simulink model "AutoSarNm"  (R2022b)
settings: Solver=FixedStepDiscrete  StartTime=0.0  StopTime=inf  FixedStep=0.01  RelTol=1e-3
PreLoadFcn:
  | canMessageBusType;
  | canFDMessageBusType;
values from neighbouring files (symbols this model uses):
  AUROSAR_NM_CANWAKEUP_ENABLE = 1.0    [AutoSarNm.sldd]
  AUROSAR_NM_MODEL_RUN_STEP = 10.0    [AutoSarNm.sldd]
  AUROSAR_NM_RDY2SLP_ENABLE = 0.0    [AutoSarNm.sldd]
  AUROSAR_NM_UDS_OVERTIME = 5000.0    [AutoSarNm.sldd]
  CAN_ID_VEH_RX_NM = 418316033    [AutoSarNm.sldd]
  CAN_ID_VEH_TX_NM = 536870910.0    [AutoSarNm.sldd]
  CANNM_BSM_WAITSLP_TIME = 500.0    [AutoSarNm.sldd]
  CANNM_IMMEDIATE_CYCLE_TIME = 20.0    [AutoSarNm.sldd]
  CANNM_IMMEDIATE_TRANSMISSION_COUNT = 10.0    [AutoSarNm.sldd]
  CANNM_MSG_CYCLE_TIME = 1000.0    [AutoSarNm.sldd]
  CANNM_NM_TIMEOUT_TIME = 2500.0    [AutoSarNm.sldd]
  CANNM_REPEAT_MEG_TIME = 3300.0    [AutoSarNm.sldd]
  CANNM_WAIT_BUS_SLEEP_TIME = 1500.0    [AutoSarNm.sldd]
libraries: simulink x7, canfdmsglib x2
PreSaveFcn:
  | filename = 'AutoSarNm';
  | dictionaryObj  = Simulink.data.dictionary.open([filename,'.sldd']);
  | saveChanges(dictionaryObj);
  | close(dictionaryObj);
  | disp([filename,'.sldd 已保存']);
settings Model: DataDictionary=AutoSarNm.sldd  Creator=Ligoo  LastModifiedBy=CASTORICE
settings DataIOCC: SaveOutput=off  SignalLogging=off  DSMLogging=off  SaveTime=off  ReturnWorkspaceOutputs=off
settings OptimizationCC: DefaultParameterBehavior=Inlined  DefaultUnderspecifiedDataType=single  EnableMemcpy=off  ActiveStateOutputEnumStorageType=uint16  ZeroExternalMemoryAtStartup=off  ZeroInternalMemoryAtStartup=off  NoFixptDivByZeroProtection=on  EfficientFloat2IntCast=on  LifeSpan=Inf  MaxStackSize=200  OptimizeBlockOrder=speed  DifferentSizesBufferReuse=on  EfficientTunableParamExpr=on
settings DebuggingCC: SignalInfNanChecking=error  SignalRangeChecking=warning  AlgebraicLoopMsg=error  MergeDetectMultiDrivingBlocksExec=none  TasksWithSamePriorityMsg=error  IntegerOverflowMsg=error  UnconnectedInputMsg=error  UnconnectedOutputMsg=error  UnconnectedLineMsg=error  UniqueDataStoreMsg=warning  ModelReferenceIOMsg=error  ModelReferenceVersionMismatchMessage=error  StateNameClashWarn=warning  SFUnexpectedBacktrackingDiag=warning  SFNoUnconditionalDefaultTransitionDiag=warning  SFUndirectedBroadcastEventsDiag=error  IntegerSaturationMsg=error
settings HardwareCC: ProdBitPerPointer=32  ProdBitPerSizeT=32  ProdBitPerPtrDiffT=32  ProdLargestAtomicInteger=Long  ProdWordSize=32  ProdLongLongMode=on  ProdHWDeviceType=ARM Compatible->ARM 7
settings ModelReferenceCC: EnableRefExpFcnMdlSchedulingChecks=on
settings SFSimCC: SimCustomHeaderCode="#include \"NMmain.h\""  SimUserSources=NMmain.c  MATLABDynamicMemAlloc=off
settings RTWCC: Description=Embedded Coder  SystemTargetFile=ert.tlc  GenCodeOnly=on  TemplateMakefile=ert_default_tmf  GenerateReport=on  RTWUseSimCustomCode=on  CustomHeaderCode="#include \"NMmain.h\""  CustomSource=NMmain.c  Toolchain=LCC-win64 v2.4.1 | gmake (64-bit Windows)  IncludeHyperlinkInReport=on  LaunchReport=on  GenerateTraceInfo=on  GenerateTraceReport=on  GenerateTraceReportSl=on  GenerateTraceReportSf=on  GenerateTraceReportEml=on
settings CodeAppCC: ForceParamTrailComments=on  IgnoreCustomStorageClasses=off  OperatorAnnotations=on  SimulinkDataObjDesc=on  SFDataObjDesc=on  MATLABFcnDesc=on  CustomSymbolStrUtil=$R$N$C  InsertBlockDesc=on  MATLABSourceComments=on
settings ERTTargetCC: MultiwordLength=2048  ConcurrentExecutionCompliant=off  IncludeMdlTerminateFcn=off  SuppressErrorStatus=on  SupportAbsoluteTime=off  SupportNonFinite=off  SupportComplex=off  ModelStepFunctionPrototypeControlCompliant=off  CPPClassGenCompliant=off  ArrayLayout=Row-major  GenerateASAP2=on  InlinedParameterPlacement=NonHierarchical  ERTCustomFileTemplate=example_file_process.tlc
settings ConfigComp: CovSaveCumulativeToWorkspaceVar=on  CovSaveSingleToWorkspaceVar=on  CovExternalEMLEnable=off  DVTestSuiteOptimization=CombinedObjectives (Nonlinear Extended)  DVDetectActiveLogic=on  DVModelReferenceHarness=on  DVHarnessSource=Signal Editor

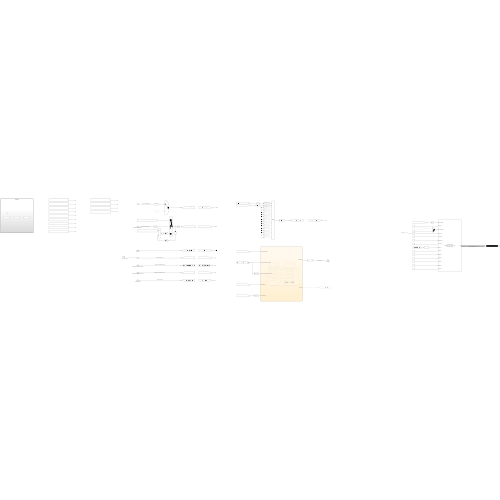
[thumbnail: Simulink's stored preview of the top-level diagram]
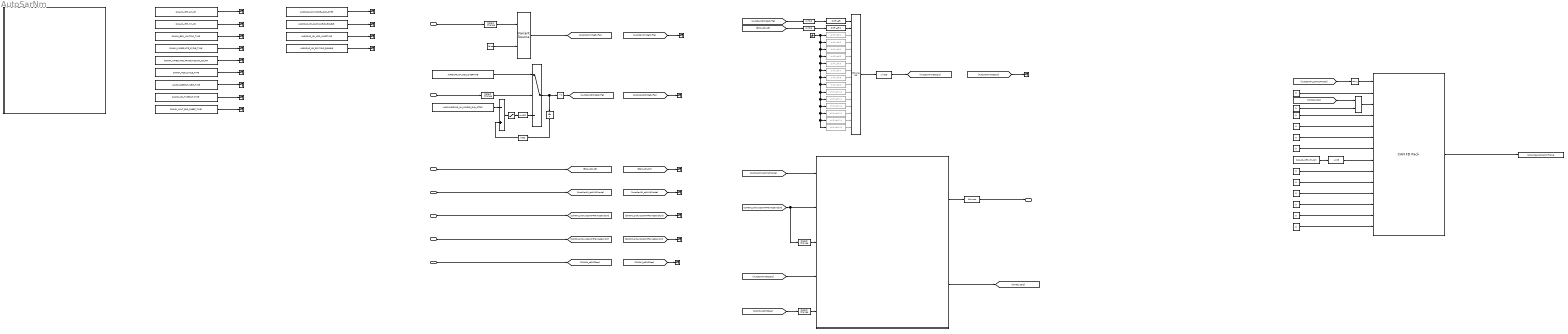
== system AutoSarNm ==
  note: 0:被动唤醒
      | 1:主动唤醒
      | 0xFF:未探测到唤醒源
  note: 分段网络管理，不支持
  AutoSarNM_cntNmMsgRxCnt : Inport
  AutoSarNM_cntUDSMsgRxCnt : Inport  Port=2
  BSW_stKL15 : Inport  Port=3
  AutoSarNM_stWKUPMode : Inport  Port=4
  CANNM_cntAuroSarNMFrameSendCnt : Inport  Port=5
  CANNM_cntAuroSarNMFrameRecvCnt : Inport  Port=6
  CANNM_stRMSReq : Inport  Port=7
  Add : Sum  Inputs=-+  OutDataTypeStr=int32
  Bitwise OR : simulink/Logic and Bit Operations/Bitwise Operator  logicop=OR  UseBitMask=off  NumInputPorts=16  BitMask=bin2dec('11011001')  BitMaskRealWorld=Stored Integer
      settings: LibrarySourceBlock=|
      | simulink/Quick Insert/Logic and Bit
      | Operations/Bitwise OR
  CAN FD Pack : canfdmsglib/CAN FD Pack  MsgList=(none)  MsgName=AutoSarNM  ProtocolMode=CAN FD  MsgIDType=Extended (29-bit identifier)  MsgIdentifier=CAN_ID_VEH_TX_NM  MsgLength=8  Remote=off  BRSSwitch=on  ApplyMinMax=off  SignalInfo={ 'CBV_ActWKUP', '12', '1', 'BE', 'unsigned', 'Standard', '0', '1', '0', '-Inf', 'Inf'; 'CBV_CID', '9', '2', 'BE', 'unsigned', 'Standard', '0', '1', '0', '-Inf', 'Inf'; 'CBV_NmSlpRdy', '11', '1', 'BE', 'unsigned', 'Standard', '0', '1', '0', '-Inf', 'Inf'; 'CBV_PNI', '14', '1', 'BE', 'unsigned', 'Standard', '0', '1', '0', '-Inf', 'Inf'; 'CBV_RESV_1', '13', '1', 'BE', 'unsigned', 'Standard', '0', '1', '0', '-Inf', 'Inf'; 'CBV_RESV_2', '15', '1', 'BE', 'unsigned', 'Standard', '0', '1', '0', '-Inf', 'Inf'; 'CBV_RMR', '8', '1', 'BE', 'unsigned', 'Standard', '0', '1', '0', '-Inf', 'Inf'; 'SourceID', '0', '8', 'BE', 'unsigned', 'Standard', '0', '1', '0', '-Inf', 'Inf'; 'UseData1', '16', '8', 'BE', 'unsigned', 'Standard', '0', '1', '0', '-Inf', 'Inf'; 'UseData2', '24', '8', 'BE', 'unsigned', 'Standard', '0', '1', '0', '-Inf', 'Inf'; 'UseData3', '32', '8', 'BE', 'unsigned', 'Standard', '0', '1', '0', '-Inf', 'Inf'; 'UseData4', '40', '8', 'BE', 'unsigned', 'Standard', '0', '1', '0', '-Inf', 'Inf'; 'UseData5', '48', '8', 'BE', 'unsigned', 'Standard', '0', '1', '0', '-Inf', 'Inf'; 'UseData6', '56', '8', 'BE', 'unsigned', 'Standard', '0', '1', '0', '-Inf', 'Inf' }
      settings: DataFormat=manually specified signals
  Chart : Stateflow chart  TreatAsAtomicUnit=on
  Compare To Constant : simulink/Logic and Bit Operations/Compare To Constant  relop=~=  const=uint32(0)  OutDataTypeStr=boolean
  Compare To Constant1 : simulink/Logic and Bit Operations/Compare To Constant  relop===  const=1  OutDataTypeStr=uint8
  Constant : Constant  Value=AUROSAR_NM_CANWAKEUP_ENABLE
  Constant1 : Constant  Value=AUROSAR_NM_MODEL_RUN_STEP
  Constant{9..12,14..20,29} (12 alike) : Constant  Value=0  OutDataTypeStr=uint8
  Constant13 : Constant  Value=AUROSAR_NM_RDY2SLP_ENABLE
  Constant2 : Constant  Value=false  OutDataTypeStr=boolean
  Constant21 : Constant  Value=CAN_ID_VEH_TX_NM
  Constant22 : Constant  Value=CANNM_BSM_WAITSLP_TIME
  Constant23 : Constant  Value=CANNM_IMMEDIATE_CYCLE_TIME
  Constant24 : Constant  Value=CANNM_IMMEDIATE_TRANSMISSION_COUNT
  Constant25 : Constant  Value=CANNM_MSG_CYCLE_TIME
  Constant26 : Constant  Value=CANNM_REPEAT_MEG_TIME
  Constant27 : Constant  Value=CANNM_NM_TIMEOUT_TIME
  Constant28 : Constant  Value=CANNM_WAIT_BUS_SLEEP_TIME
  Constant3 : Constant  Value=AUROSAR_NM_UDS_OVERTIME
  Constant4 : Constant  Value=AUROSAR_NM_UDS_OVERTIME
  Constant5 : Constant  Value=int32(AUROSAR_NM_MODEL_RUN_STEP)
  Constant7 : Constant  Value=CAN_ID_VEH_RX_NM
  Constant8 : Constant  Value=CAN_ID_VEH_TX_NM  OutDataTypeStr=uint32
  Data Store Write : DataStoreWrite  DataStoreName=CAN_msgAutoSarNmFrame  IndexOptions=Index vector (dialog)  Indices=1  OutputSizes=1
  Data Type Conversion : DataTypeConversion  OutDataTypeStr=uint16  SaturateOnIntegerOverflow=off  RndMeth=Floor
  Data Type Conversion1 : DataTypeConversion  OutDataTypeStr=Enum: AutoSarNm_Sts_Enum  SaturateOnIntegerOverflow=off  RndMeth=Floor
  Data Type Conversion2 : DataTypeConversion  OutDataTypeStr=uint16  SaturateOnIntegerOverflow=off  RndMeth=Floor
  Data Type Conversion3 : DataTypeConversion  OutDataTypeStr=uint16  SaturateOnIntegerOverflow=off  RndMeth=Floor
  Data Type Conversion4 : DataTypeConversion  OutDataTypeStr=int32  SaturateOnIntegerOverflow=off  RndMeth=Floor
  Data Type Conversion5 : DataTypeConversion  OutDataTypeStr=uint32  SaturateOnIntegerOverflow=off  RndMeth=Floor
  Data Type Conversion6 : DataTypeConversion  OutDataTypeStr=uint8  SaturateOnIntegerOverflow=off  RndMeth=Floor
  Detect Change : simulink/Logic and Bit Operations/Detect Change  vinit=0  OutDataTypeStr=boolean
  Detect Change1 : simulink/Logic and Bit Operations/Detect Change  vinit=0  OutDataTypeStr=boolean
  Detect Change2 : simulink/Logic and Bit Operations/Detect Change  vinit=0  OutDataTypeStr=uint8
  Detect Change3 : simulink/Logic and Bit Operations/Detect Change  vinit=0  OutDataTypeStr=uint8
  Ground : Ground
  Initialize Function : Subsystem  TreatAsAtomicUnit=on
  Saturation : Saturate  UpperLimit=int32(AUROSAR_NM_UDS_OVERTIME)  LowerLimit=0
  Shift Arithmetic : ArithShift  BitShiftDirection=Left
  Shift Arithmetic1 : ArithShift  BitShiftNumber=1  BitShiftDirection=Left
  Shift Arithmetic10 : ArithShift  Commented=on  BitShiftNumber=10  BitShiftDirection=Left
  Shift Arithmetic11 : ArithShift  Commented=on  BitShiftNumber=11  BitShiftDirection=Left
  Shift Arithmetic12 : ArithShift  Commented=on  BitShiftNumber=12  BitShiftDirection=Left
  Shift Arithmetic13 : ArithShift  Commented=on  BitShiftNumber=13  BitShiftDirection=Left
  Shift Arithmetic14 : ArithShift  Commented=on  BitShiftNumber=14  BitShiftDirection=Left
  Shift Arithmetic15 : ArithShift  Commented=on  BitShiftNumber=15  BitShiftDirection=Left
  Shift Arithmetic2 : ArithShift  Commented=on  BitShiftNumber=2  BitShiftDirection=Left
  Shift Arithmetic3 : ArithShift  Commented=on  BitShiftNumber=3  BitShiftDirection=Left
  Shift Arithmetic4 : ArithShift  Commented=on  BitShiftNumber=4  BitShiftDirection=Left
  Shift Arithmetic5 : ArithShift  Commented=on  BitShiftNumber=5  BitShiftDirection=Left
  Shift Arithmetic6 : ArithShift  Commented=on  BitShiftNumber=6  BitShiftDirection=Left
  Shift Arithmetic7 : ArithShift  Commented=on  BitShiftNumber=7  BitShiftDirection=Left
  Shift Arithmetic8 : ArithShift  Commented=on  BitShiftNumber=8  BitShiftDirection=Left
  Shift Arithmetic9 : ArithShift  Commented=on  BitShiftNumber=9  BitShiftDirection=Left
  Switch : Switch  Criteria=u2 > Threshold  SaturateOnIntegerOverflow=off  InputSameDT=off
  Terminator{,1..20} (21 alike) : Terminator
  Unit Delay : UnitDelay  SampleTime=-1  HasFrameUpgradeWarning=on
  Variant Source : VariantSource  VariantActivationTime=code compile
  Variant Source1 : VariantSource  VariantActivationTime=code compile
  AutoSarNM_sts : Outport
  wires:
  Constant/1 -> Terminator/1
  AutoSarNM_cntNmMsgRxCnt/1 -> Detect Change/1  "AutoSarNM_cntNmMsgRxCnt"
  Constant1/1 -> Terminator1/1
  Detect Change/1 -> Variant Source/1
  Constant2/1 -> Variant Source/2
  Variant Source/1 -> [AutoSarNmMsgRxFlg]
  [AutoSarNmMsgRxFlg] -> Terminator2/1
  AutoSarNM_cntUDSMsgRxCnt/1 -> Detect Change1/1  "AutoSarNM_cntUDSMsgRxCnt"
  Constant3/1 -> Terminator3/1
  Detect Change1/1 -> Switch/2
  Constant4/1 -> Switch/1
  Add/1 -> Saturation/1
  Switch/1 -> Compare To Constant/1, Unit Delay/1
  Unit Delay/1 -> Data Type Conversion4/1
  Constant5/1 -> Add/1
  Saturation/1 -> Data Type Conversion5/1
  Compare To Constant/1 -> [AutoSarUDSMsgRxFlg]
  [AutoSarUDSMsgRxFlg] -> Terminator4/1
  [AutoSarUDSMsgRxFlg] -> Data Type Conversion2/1
  BSW_stKL15/1 -> [BSW_stKL15]  "BSW_stKL15"
  [BSW_stKL15] -> Terminator5/1
  Shift Arithmetic/1 -> Bitwise OR/1
  Bitwise OR/1 -> Data Type Conversion/1
  [BSW_stKL15] -> Data Type Conversion3/1
  Shift Arithmetic1/1 -> Bitwise OR/2
  Ground/1 -> Shift Arithmetic15/1, Shift Arithmetic14/1, Shift Arithmetic13/1, Shift Arithmetic12/1, Shift Arithmetic11/1, Shift Arithmetic10/1, Shift Arithmetic9/1, Shift Arithmetic8/1, Shift Arithmetic7/1, Shift Arithmetic6/1, Shift Arithmetic5/1, Shift Arithmetic4/1, Shift Arithmetic3/1, Shift Arithmetic2/1
  Shift Arithmetic2/1 -> Bitwise OR/3
  Shift Arithmetic3/1 -> Bitwise OR/4
  Shift Arithmetic4/1 -> Bitwise OR/5
  Shift Arithmetic5/1 -> Bitwise OR/6
  Shift Arithmetic6/1 -> Bitwise OR/7
  Shift Arithmetic7/1 -> Bitwise OR/8
  Shift Arithmetic8/1 -> Bitwise OR/9
  Shift Arithmetic9/1 -> Bitwise OR/10
  Shift Arithmetic10/1 -> Bitwise OR/11
  Shift Arithmetic11/1 -> Bitwise OR/12
  Shift Arithmetic12/1 -> Bitwise OR/13
  Shift Arithmetic13/1 -> Bitwise OR/14
  Shift Arithmetic14/1 -> Bitwise OR/15
  Shift Arithmetic15/1 -> Bitwise OR/16
  Data Type Conversion/1 -> [AutoSarNmKeepSrc]
  [AutoSarNmKeepSrc] -> Terminator6/1
  Constant7/1 -> Terminator7/1
  Constant8/1 -> Data Type Conversion6/1
  Constant9/1 -> CAN FD Pack/4
  Constant10/1 -> CAN FD Pack/5
  Constant11/1 -> CAN FD Pack/6
  Constant12/1 -> CAN FD Pack/7
  AutoSarNM_stWKUPMode/1 -> [AutoSarNM_stWKUPMode]  "AutoSarNM_stWKUPMode"
  Constant14/1 -> CAN FD Pack/2
  Constant15/1 -> CAN FD Pack/9
  Constant16/1 -> CAN FD Pack/10
  Constant17/1 -> CAN FD Pack/11
  Constant18/1 -> CAN FD Pack/12
  Constant19/1 -> CAN FD Pack/13
  Constant20/1 -> CAN FD Pack/14
  Constant21/1 -> Terminator8/1
  Constant22/1 -> Terminator9/1
  [AutoSarNM_stWKUPMode] -> Terminator10/1
  [AutoSarNM_stWKUPMode] -> Compare To Constant1/1
  Compare To Constant1/1 -> CAN FD Pack/1
  [AutoSarNM_stWKUPMode] -> Chart/1(AutoSarNM_stWKUPMode)
  Constant23/1 -> Terminator11/1
  CANNM_cntAuroSarNMFrameSendCnt/1 -> [CANNM_cntAuroSarNMFrameSendCnt]  "CANNM_cntAuroSarNMFrameSendCnt"
  [CANNM_cntAuroSarNMFrameSendCnt] -> Terminator12/1
  [CANNM_cntAuroSarNMFrameSendCnt] -> Detect Change3/1, Chart/2(CANNM_cntAuroSarNMFrameSendCnt)
  Constant24/1 -> Terminator13/1
  CANNM_cntAuroSarNMFrameRecvCnt/1 -> [CANNM_cntAuroSarNMFrameRecvCnt]  "CANNM_cntAuroSarNMFrameRecvCnt"
  [CANNM_cntAuroSarNMFrameRecvCnt] -> Terminator14/1
  Constant25/1 -> Terminator15/1
  [AutoSarNmKeepSrc] -> Chart/4(AutoSarNmKeepSrc)
  Constant26/1 -> Terminator16/1
  Chart/1(AutoSarNM_sts) -> Data Type Conversion1/1
  CANNM_stRMSReq/1 -> [CANNM_stRMSReq]  "CANNM_stRMSReq"
  [CANNM_stRMSReq] -> Terminator17/1
  [CANNM_stRMSReq] -> Detect Change2/1
  Detect Change2/1 -> Chart/5(CANNM_stRMSReq)
  Constant27/1 -> Terminator18/1
  Constant28/1 -> Terminator19/1
  Chart/2(NmRdy2Slp) -> [NmRdy2Slp]
  Data Type Conversion1/1 -> AutoSarNM_sts/1  "AutoSarNM_sts"
  Data Type Conversion2/1 -> Shift Arithmetic/1
  Data Type Conversion3/1 -> Shift Arithmetic1/1
  Data Type Conversion4/1 -> Add/2
  Data Type Conversion5/1 -> Switch/3
  CAN FD Pack/1 -> Data Store Write/1  "CAN_msgAutoSarNmFrame"
  Data Type Conversion6/1 -> CAN FD Pack/8
  Detect Change3/1 -> Chart/3(CANNM_cntAuroSarNMFrameSendCnt_Step)
  Constant13/1 -> Terminator20/1
  Variant Source1/1 -> CAN FD Pack/3
  [NmRdy2Slp] -> Variant Source1/1
  Constant29/1 -> Variant Source1/2

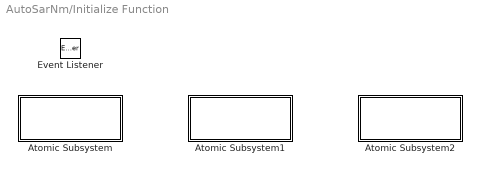
== system AutoSarNm/Initialize Function ==
  Atomic Subsystem : Subsystem  Priority=1  TreatAsAtomicUnit=on
  Atomic Subsystem1 : Subsystem  Priority=2  TreatAsAtomicUnit=on
  Atomic Subsystem2 : Subsystem  Priority=3  TreatAsAtomicUnit=on
  Event Listener : EventListener  DisableCoverage=on  EventName=reset

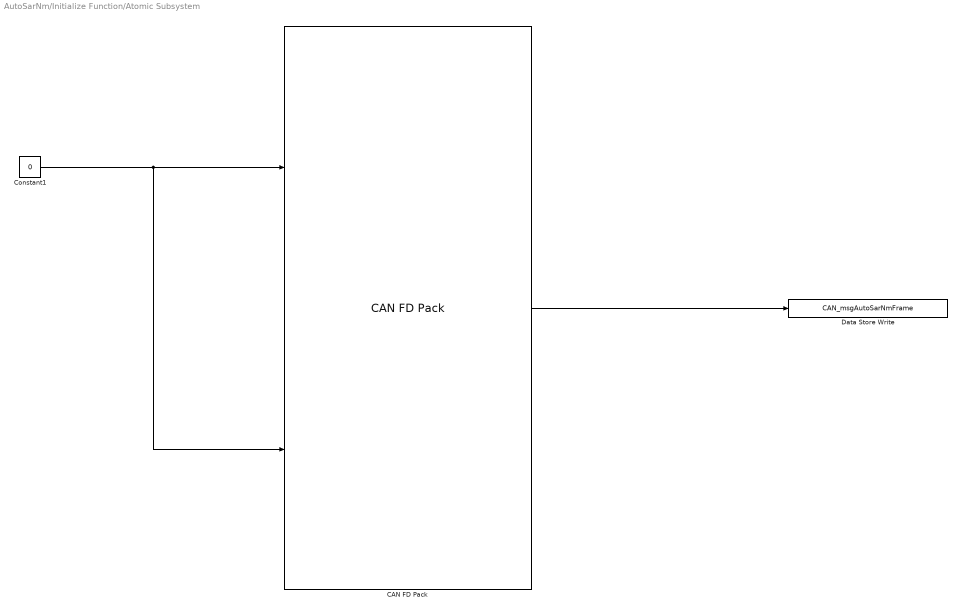
== system AutoSarNm/Initialize Function/Atomic Subsystem ==
  CAN FD Pack : canfdmsglib/CAN FD Pack  MsgList=(none)  MsgName=AutoSarNM  ProtocolMode=CAN FD  MsgIDType=Extended (29-bit identifier)  MsgIdentifier=CAN_ID_VEH_TX_NM  MsgLength=8  Remote=off  BRSSwitch=on  ApplyMinMax=off  SignalInfo={ 'Signal1', '0', '32', 'LE', 'signed', 'Standard', '0', '1', '0', '-Inf', 'Inf'; 'Signal2', '32', '32', 'LE', 'signed', 'Standard', '0', '1', '0', '-Inf', 'Inf' }
      settings: DataFormat=manually specified signals
  Constant1 : Constant  Value=0  OutDataTypeStr=uint8
  Data Store Write : DataStoreWrite  DataStoreName=CAN_msgAutoSarNmFrame  IndexOptions=Index vector (dialog)  Indices=1  OutputSizes=1
  wires:
  CAN FD Pack/1 -> Data Store Write/1
  Constant1/1 -> CAN FD Pack/2, CAN FD Pack/1

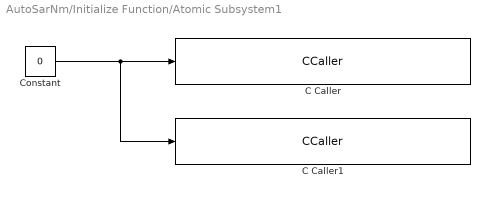
== system AutoSarNm/Initialize Function/Atomic Subsystem1 ==
  C Caller : CCaller  FunctionName=NM_SetAppMsgEnable  PortSpecificationStruct="%)30     .    * (   8    (     @         %    \"     $    !     0         %  0 \"0    $    _    07)G3F%M90  4&]R=$YA;64 4V-O<&4     26YD97@     5'EP90      4VEZ90      27-';&]B86P   X    X    !@    @    $          4    (     0    8    !         !     &    16YA8FQE   .    .     8    (    !          %    \"     $    &     0         0    !@   $5N86)L90  #@   #@    &    \"     0         !0    @    !    !0    $         $     4   !);G!U=     X    X    !@    @    &          4    (     0    $    !          D    (               .    .     8    (    !          %    \"     $    %     0         0    !0   '5I;G0X    #@   #     &    \"     0         !0    @    !     0    $         $  ! #$    .    ,     8    (    \"0(        %    \"     $    !     0         \"  $"
  C Caller1 : CCaller  FunctionName=NM_SetNmMsgEnable  PortSpecificationStruct="%)30     .    * (   8    (     @         %    \"     $    !     0         %  0 \"0    $    _    07)G3F%M90  4&]R=$YA;64 4V-O<&4     26YD97@     5'EP90      4VEZ90      27-';&]B86P   X    X    !@    @    $          4    (     0    8    !         !     &    16YA8FQE   .    .     8    (    !          %    \"     $    &     0         0    !@   $5N86)L90  #@   #@    &    \"     0         !0    @    !    !0    $         $     4   !);G!U=     X    X    !@    @    &          4    (     0    $    !          D    (               .    .     8    (    !          %    \"     $    %     0         0    !0   '5I;G0X    #@   #     &    \"     0         !0    @    !     0    $         $  ! #$    .    ,     8    (    \"0(        %    \"     $    !     0         \"  $"
  Constant : Constant  Value=0  OutDataTypeStr=uint8
  wires:
  Constant/1 -> C Caller1/1, C Caller/1

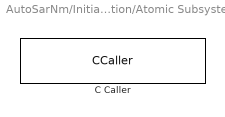
== system AutoSarNm/Initialize Function/Atomic Subsystem2 ==
  C Caller : CCaller  FunctionName=NM_BsmGetWkupMode

== stateflow chart AutoSarNm/Chart ==
  state BSM
    en:
    NM_SetNmMsgEnable(uint8(0));
    NM_SetAppMsgEnable(uint8(0));
    NM_ResetCanNmSendCnt();
    App_SendFlg = 0;
    AutoSarNM_sts = uint8(0);
    NmRdy2Slp = 0;
    NM_PbsmGetWkupMode(uint8(1));
    du:
    NM_PbsmGetWkupMode(uint8(0));
    state wait
    state wait1
      en:
      NM_EnterSleepMode();
    (default) -> BSM.wait
    BSM.wait -> wait1 : [after(CANNM_BSM_WAITSLP_TIME,msec)]
  state PBSM
    en:
    AutoSarNM_sts = uint8(1);
    NM_SetAppMsgEnable(uint8(0));
    NM_ResetCanNmSendCnt();
    NM_ResetWKUPMode();
    App_SendFlg = 0;
    NM_PbsmGetWkupMode(uint8(1));
    du:
    NM_PbsmGetWkupMode(uint8(0));
  state ALL
    state RMS
      en:
      AutoSarNM_sts = uint8(2);
      %1、上电后首帧必须是网管管理帧
      %2、被动唤醒不进入快发模式
      state Set_AppSendMode [parallel]
        settings: executionOrder=1
        state Fast
        state Slow
          en:
          NM_SetAppMsgEnable(uint8(1));
          App_SendFlg = 1;
        (default) -> ALL.RMS.Set_AppSendMode.Fast [order 1] : [App_SendFlg == 0]
        (default) -> ALL.RMS.Set_AppSendMode.Slow [order 2]
        ALL.RMS.Set_AppSendMode.Fast -> ALL.RMS.Set_AppSendMode.Slow : [CANNM_cntAuroSarNMFrameSendCnt > 0]
      state Set_NmSendMode [parallel]
        settings: executionOrder=2
        state Slow
          en:
          NM_SetNmMsgEnable(uint8(1));
          NM_SetNmMsgCycle(CANNM_MSG_CYCLE_TIME);
        state Fast
          en:
          NM_SetNmMsgCycle(CANNM_IMMEDIATE_CYCLE_TIME);
          NM_SetNmMsgEnable(uint8(1));
          NM_ResetCanNmSendCnt();
          RMSSendFrameCntDelay = CANNM_cntAuroSarNMFrameSendCnt;
        (default) -> ALL.RMS.Set_NmSendMode.Slow [order 2]
        (default) -> ALL.RMS.Set_NmSendMode.Fast [order 1] : [AutoSarNM_stWKUPMode == 0 || CANNM_stRMSReq ~= 0]
        ALL.RMS.Set_NmSendMode.Fast -> ALL.RMS.Set_NmSendMode.Slow : [CANNM_cntAuroSarNMFrameSendCnt - RMSSendFrameCntDelay >= CANNM_IMMEDIATE_TRANSMISSION_COUNT]
    state NOS
      en:
      AutoSarNM_sts = uint8(3);
    state RSS
      en:
      AutoSarNM_sts = uint8(4);
      state SendLastFrame [parallel]
        settings: executionOrder=1
        state wait
          en:
          NmRdy2Slp = 1;
          RMSSendFrameCntDelay = CANNM_cntAuroSarNMFrameSendCnt;
        state end
          en:
          NmRdy2Slp = 0;
          NM_SetNmMsgEnable(uint8(0));
        (default) -> ALL.RSS.SendLastFrame.wait [order 1] : [AUROSAR_NM_RDY2SLP_ENABLE ~= 0]
        ALL.RSS.SendLastFrame.wait -> end : [RMSSendFrameCntDelay ~= CANNM_cntAuroSarNMFrameSendCnt]
        (default) -> end [order 2]
      state OverTime [parallel]
        settings: executionOrder=2
        state wait_
        (default) -> wait_
        wait_ -> wait_ [order 2] : [CANNM_cntAuroSarNMFrameSendCnt_Step ~= 0]
    RMS -> (junction 36) : [after(CANNM_REPEAT_MEG_TIME,msec)]
    (junction 36) -> NOS [order 1] : [AutoSarNmKeepSrc ~= 0]
    (junction 36) -> RSS [order 2]
    RSS -> NOS : [AutoSarNmKeepSrc ~= 0]
        | {NM_SetNmMsgEnable(uint8(1));}
    NOS -> RSS : [AutoSarNmKeepSrc == 0]
  wait_ -> PBSM [order 1] : [after(CANNM_NM_TIMEOUT_TIME,msec)]
  (default) -> BSM
  PBSM -> wait1 [order 2] : [after(CANNM_WAIT_BUS_SLEEP_TIME,msec)]
  BSM -> RMS : [AutoSarNM_stWKUPMode ~= hex2dec('0xFF')]
  PBSM -> RMS [order 1] : [AutoSarNM_stWKUPMode ~= hex2dec('0xFF')]
  ALL -> (junction 63) : [CANNM_stRMSReq ~= 0]
  (junction 63) -> (junction 65)
  (junction 65) -> ALL.RMS.Set_NmSendMode.Fast
  data: CANNM_BSM_WAITSLP_TIME parameter; AutoSarNM_stWKUPMode input; CANNM_IMMEDIATE_CYCLE_TIME parameter; CANNM_cntAuroSarNMFrameSendCnt input; CANNM_cntAuroSarNMFrameSendCnt_Step input; App_SendFlg local uint8; AutoSarNmKeepSrc input; CANNM_MSG_CYCLE_TIME parameter; CANNM_REPEAT_MEG_TIME parameter; AutoSarNM_sts output; RMSSendFrameCntDelay local uint32; CANNM_stRMSReq input; CANNM_NM_TIMEOUT_TIME parameter; CANNM_WAIT_BUS_SLEEP_TIME parameter; NmRdy2Slp output uint8; CANNM_IMMEDIATE_TRANSMISSION_COUNT parameter; AUROSAR_NM_RDY2SLP_ENABLE parameter
